simulink model "pfb_fft_d3a"  (R2021a)
settings: Solver=VariableStepAuto  StartTime=0.0  StopTime=100.0  RelTol=1e-3
undefined symbols (not defined in the file): i, pfb_coeff_gen_calc
libraries: xbsIndex_r4 x11529, casper_library_misc x39, casper_library_delays x39, xbsReplacements_r4 x2
(part 40 of 118)

== system pfb_fft_d3a/fft_wideband_real/fft_biplex_real_4x/biplex_core/fft_stage_10/butterfly_direct ==
  a : Inport
  b : Inport  Port=2
  sync_in : Inport  Port=3
  shift : Inport  Port=4
  Concat : xbsIndex_r4/Concat  num_inputs=2  dbl_ovrd=off  block_type=concat
  bus_add : Subsystem  AncestorBlock=casper_library_bus/bus_addsub  mask(bus_addsub){opmode=0, n_bits_a=[18 18], bin_pt_a=17, type_a=1, n_bits_b=[19 19], bin_pt_b=17, type_b=1, cmplx=on, misc=off, async=off, floating_point=off, float_type=single, exp_width=8, frac_width=24, n_bits_out=20, bin_pt_out=17, type_out=1, quantization=0, overflow=0, add_implementation=behavioral HDL, csp_latency=1, pipeline_en=off, pipeline_latency=0}
      mask prompts: opmode "mode (Addition=0, Subtraction=1)"; n_bits_a "a input bit widths"; bin_pt_a "a input binary points"; type_a "a input type (Unsigned=0, Signed=1)"; n_bits_b "b input bit widths"; bin_pt_b "b input binary points"; type_b "b input type (Unsigned=0, Signed=1)"; cmplx "complex"; misc "misc support"; async "asynchronous operation"; floating_point "floating point"; exp_width "exponent width"; frac_width "fraction width"; n_bits_out "output bit widths"; bin_pt_out "output binary points"; type_out "output type (Unsigned=0, Signed=1)"; quantization "quantization strategy (Truncate=0, Round  (unbiased: +/- Inf)=1)"; overflow "overflow strategy (Wrap=0, Saturate=1, Flag as error=2)"; add_implementation "adder implementation"; csp_latency "latency"; pipeline_en "pipeline enable"; pipeline_latency "pipeline latency"
      mask help: Add/subtract components of two busses
      mask init: same as pfb_fft_d3a/fft_wideband_real/fft_direct/butterfly0_0/bus_add
      mask Callback floating_point:
      | onoff = get_param(gcb, 'floating_point');
      | if strcmp(onoff,'on')
      |     enable_fixpt = 'off';
      |     set_param_state(gcb, 'float_type', 'on')
      | 
      |     f_type = get_param(gcb, 'float_type');
      |     if strcmp(f_type,'custom')
      |         set_param_state(gcb, 'exp_width', 'on')
      |         set_param_state(gcb, 'frac_width', 'on')
      |     else
      |         set_param_state(gcb, 'exp_width', 'off')
      |         set_param_state(gcb, 'frac_width', 'off')
      |     end
      | 
      | 
      | else
      |     enable_fixpt = 'on';
      |     set_param_state(gcb, 'float_type', 'off')
      |     set_param_state(gcb, 'exp_width', 'off')
      |     set_param_state(gcb, 'frac_width', 'off')
      | end
      | 
      | set_param_state(gcb, 'n_bits_a', enable_fixpt)
      | set_param_state(gcb, 'bin_pt_a', enable_fixpt)
      | set_param_state(gcb, 'type_a', enable_fixpt)
      | set_param_state(gcb, 'n_bits_b', enable_fixpt)
      | set_param_state(gcb, 'bin_pt_b', enable_fixpt)
      | set_param_state(gcb, 'type_b', enable_fixpt)
      | 
      | set_param_state(gcb, 'n_bits_out', enable_fixpt)
      | set_param_state(gcb, 'bin_pt_out', enable_fixpt)
      | set_param_state(gcb, 'type_out', enable_fixpt)
      | set_param_state(gcb, 'quantization', enable_fixpt)
      | set_param_state(gcb, 'overflow', enable_fixpt)
      mask TypeOptions float_type: single | custom
      mask Callback float_type:
      | f_type = get_param(gcb, 'float_type');
      | if strcmp(f_type,'custom')
      |     set_param_state(gcb, 'exp_width', 'on')
      |     set_param_state(gcb, 'frac_width', 'on')
      | else
      |     set_param_state(gcb, 'exp_width', 'off')
      |     set_param_state(gcb, 'frac_width', 'off')
      | end
      mask TypeOptions add_implementation: behavioral HDL | fabric core | DSP48 core
  bus_convert : Subsystem  AncestorBlock=casper_library_bus/bus_convert  mask(bus_convert){n_bits_in=[21 21 21 21], bin_pt_in=[18 18 18 18], cmplx=on, n_bits_out=18, bin_pt_out=17, quantization=2, overflow=0, csp_latency=conv_latency, of=on, misc=off}
      mask prompts: n_bits_in "input bit widths"; bin_pt_in "input binary points"; cmplx "input complex"; n_bits_out "output bit widths"; bin_pt_out "output binary points"; quantization "quantization strategy (Truncate=0, Round  (unbiased: +/- Inf)=1, Round (unbiased: Even Values)=2)"; overflow "overflow strategy (Wrap=0, Saturate=1, Flag as error=2)"; csp_latency "latency"; of "overflow indication"; misc "misc support"
      mask help: Convert components of busses
      mask init: same as pfb_fft_d3a/fft_wideband_real/fft_direct/butterfly0_0/bus_convert
  bus_expand : Subsystem  AncestorBlock=casper_library_flow_control/bus_expand  mask(bus_expand){mode=divisions of equal size, outputNum=2, outputWidth=[72 72], outputBinaryPt=[0,0], outputArithmeticType=[0,0], show_format=off, outputToWorkspace=off, variablePrefix=out, outputToModelAsWell=on}
      mask prompts: outputNum "Number of outputs:"; outputWidth "Output width:"; outputBinaryPt "Output binary point position:"; outputArithmeticType "Output arithmetic type (ufix=0, fix=1, bool=2):"; show_format "Print format string?"; outputToWorkspace "Output to workspace?"; variablePrefix "Variable name prefix:"; outputToModelAsWell "Output to model as well?"
      mask help:
      | Expands a 'bus' made using a bus_create or Xilinx
      | concat block.
      | The input will be divided into the specified number
      | of outputs with the specified arithmetic types.
      | Divisions are made from most significant bit.
      mask init: same as pfb_fft_d3a/fft_wideband_real/fft_biplex_real_4x/pol0_debus
      settings: AttributesFormatString=2 outputs
      mask TypeOptions mode: divisions of equal size | divisions of arbitrary size
      mask Callback mode: %bus_expand_callback();
      mask Callback outputWidth: %bus_expand_callback();
      mask Callback outputToWorkspace: %bus_expand_callback();
  bus_norm0 : Subsystem  AncestorBlock=casper_library_bus/bus_convert  mask(bus_convert){n_bits_in=[20 20 20 20], bin_pt_in=[17 17 17 17], cmplx=on, n_bits_out=21, bin_pt_out=18, quantization=0, overflow=0, csp_latency=0, of=off, misc=off}
      mask prompts: n_bits_in "input bit widths"; bin_pt_in "input binary points"; cmplx "input complex"; n_bits_out "output bit widths"; bin_pt_out "output binary points"; quantization "quantization strategy (Truncate=0, Round  (unbiased: +/- Inf)=1, Round (unbiased: Even Values)=2)"; overflow "overflow strategy (Wrap=0, Saturate=1, Flag as error=2)"; csp_latency "latency"; of "overflow indication"; misc "misc support"
      mask help: Convert components of busses
      mask init: same as pfb_fft_d3a/fft_wideband_real/fft_direct/butterfly0_0/bus_convert
  bus_norm1 : Subsystem  AncestorBlock=casper_library_bus/bus_convert  mask(bus_convert){n_bits_in=[20 20 20 20], bin_pt_in=[18 18 18 18], cmplx=on, n_bits_out=21, bin_pt_out=18, quantization=0, overflow=0, csp_latency=0, of=off, misc=off}
      mask prompts: n_bits_in "input bit widths"; bin_pt_in "input binary points"; cmplx "input complex"; n_bits_out "output bit widths"; bin_pt_out "output binary points"; quantization "quantization strategy (Truncate=0, Round  (unbiased: +/- Inf)=1, Round (unbiased: Even Values)=2)"; overflow "overflow strategy (Wrap=0, Saturate=1, Flag as error=2)"; csp_latency "latency"; of "overflow indication"; misc "misc support"
      mask help: Convert components of busses
      mask init: same as pfb_fft_d3a/fft_wideband_real/fft_direct/butterfly0_0/bus_convert
  bus_relational : Subsystem  AncestorBlock=casper_library_bus/bus_relational  mask(bus_relational){n_bits_a=4, bin_pt_a=0, type_a=0, n_bits_b=[4 4], bin_pt_b=0, type_b=0, en=off, misc=off, mode=a!=b, csp_latency=1}
      mask prompts: n_bits_a "a input bit widths"; bin_pt_a "a input binary points"; type_a "a input type (Unsigned=0, Signed=1)"; n_bits_b "b input bit widths"; bin_pt_b "b input binary points"; type_b "b input type (Unsigned=0, Signed=1)"; en "en port"; misc "misc support"; mode "comparison:"; csp_latency "latency"
      mask help: Find the relational product of two busses
      mask init: same as pfb_fft_d3a/fft_wideband_real/fft_direct/butterfly0_0/bus_relational
      mask TypeOptions mode: a=b | a!=b | a<b | a>b | a<=b | a>=b
  bus_scale : Subsystem  AncestorBlock=casper_library_bus/bus_scale  mask(bus_scale){n_bits_in=[20 20 20 20], bin_pt_in=17, type_in=1, cmplx=on, scale_factor=-1, misc=off}
      mask prompts: n_bits_in "input bit widths"; bin_pt_in "input binary points"; type_in "input types"; cmplx "input complex"; scale_factor "scale factor (2^?)"; misc "misc support"
      mask help: Convert components of busses
      mask init:
      | bus_scale_init(gcb, ...
      |     'n_bits_in', n_bits_in, ...
      |     'bin_pt_in', bin_pt_in, ...
      |     'type_in', type_in, ...
      |     'cmplx', cmplx, ...
      |     'scale_factor', scale_factor, ...
      |     'misc', misc);
  bus_sub : Subsystem  AncestorBlock=casper_library_bus/bus_addsub  mask(bus_addsub){opmode=1, n_bits_a=[18 18], bin_pt_a=17, type_a=1, n_bits_b=[19 19], bin_pt_b=17, type_b=1, cmplx=on, misc=off, async=off, floating_point=off, float_type=single, exp_width=8, frac_width=24, n_bits_out=20, bin_pt_out=17, type_out=1, quantization=0, overflow=0, add_implementation=behavioral HDL, csp_latency=1, pipeline_en=off, pipeline_latency=0}
      mask prompts: opmode "mode (Addition=0, Subtraction=1)"; n_bits_a "a input bit widths"; bin_pt_a "a input binary points"; type_a "a input type (Unsigned=0, Signed=1)"; n_bits_b "b input bit widths"; bin_pt_b "b input binary points"; type_b "b input type (Unsigned=0, Signed=1)"; cmplx "complex"; misc "misc support"; async "asynchronous operation"; floating_point "floating point"; exp_width "exponent width"; frac_width "fraction width"; n_bits_out "output bit widths"; bin_pt_out "output binary points"; type_out "output type (Unsigned=0, Signed=1)"; quantization "quantization strategy (Truncate=0, Round  (unbiased: +/- Inf)=1)"; overflow "overflow strategy (Wrap=0, Saturate=1, Flag as error=2)"; add_implementation "adder implementation"; csp_latency "latency"; pipeline_en "pipeline enable"; pipeline_latency "pipeline latency"
      mask help: Add/subtract components of two busses
      mask init: same as pfb_fft_d3a/fft_wideband_real/fft_direct/butterfly0_0/bus_add
      mask Callback floating_point:
      | onoff = get_param(gcb, 'floating_point');
      | if strcmp(onoff,'on')
      |     enable_fixpt = 'off';
      |     set_param_state(gcb, 'float_type', 'on')
      | 
      |     f_type = get_param(gcb, 'float_type');
      |     if strcmp(f_type,'custom')
      |         set_param_state(gcb, 'exp_width', 'on')
      |         set_param_state(gcb, 'frac_width', 'on')
      |     else
      |         set_param_state(gcb, 'exp_width', 'off')
      |         set_param_state(gcb, 'frac_width', 'off')
      |     end
      | 
      | 
      | else
      |     enable_fixpt = 'on';
      |     set_param_state(gcb, 'float_type', 'off')
      |     set_param_state(gcb, 'exp_width', 'off')
      |     set_param_state(gcb, 'frac_width', 'off')
      | end
      | 
      | set_param_state(gcb, 'n_bits_a', enable_fixpt)
      | set_param_state(gcb, 'bin_pt_a', enable_fixpt)
      | set_param_state(gcb, 'type_a', enable_fixpt)
      | set_param_state(gcb, 'n_bits_b', enable_fixpt)
      | set_param_state(gcb, 'bin_pt_b', enable_fixpt)
      | set_param_state(gcb, 'type_b', enable_fixpt)
      | 
      | set_param_state(gcb, 'n_bits_out', enable_fixpt)
      | set_param_state(gcb, 'bin_pt_out', enable_fixpt)
      | set_param_state(gcb, 'type_out', enable_fixpt)
      | set_param_state(gcb, 'quantization', enable_fixpt)
      | set_param_state(gcb, 'overflow', enable_fixpt)
      mask TypeOptions float_type: single | custom
      mask Callback float_type:
      | f_type = get_param(gcb, 'float_type');
      | if strcmp(f_type,'custom')
      |     set_param_state(gcb, 'exp_width', 'on')
      |     set_param_state(gcb, 'frac_width', 'on')
      | else
      |     set_param_state(gcb, 'exp_width', 'off')
      |     set_param_state(gcb, 'frac_width', 'off')
      | end
      mask TypeOptions add_implementation: behavioral HDL | fabric core | DSP48 core
  constant : xbsIndex_r4/Constant  const=0  gui_display_data_type=Fixed-point  arith_type=Unsigned  n_bits=4  bin_pt=0  preci_type=Single  exp_width=8  frac_width=24  explicit_period=on  period=1  equ=P=C  opselect=C  inp2=PCIN>>17  opr=+  inp1=P  carry=CIN  dbl_ovrd=off  block_type=constant
  delay0 : xbsIndex_r4/Delay  rst=off  infoeditControl=Selection of Reset will increase slice count due to use of real FFs and instead of SRLs  en=off  latency=add_latency+1+conv_latency  reg_retiming=on  dbl_ovrd=off  block_type=delay
  munge : Subsystem  AncestorBlock=casper_library_flow_control/munge  mask(munge){divisions=4, div_size=[2 2 2 2], order=[0 2 1 3], arith_type_out=Unsigned, bin_pt_out=0}
      mask prompts: divisions "Number of divisions"; div_size "Division size (bits)"; order "Division packing order"; arith_type_out "Output arithmetic type"; bin_pt_out "Output binary point"
      mask help: Splits an input bus into the specified number of divisions and then recombines them in the order specified (most significant division = 0,least = number divisions-1)
      mask init:
      | munge_init(gcb, ...
      |     'divisions', divisions, ...
      |     'div_size', div_size, ...
      |     'order', order, ...
      |     'arith_type_out', arith_type_out, ...
      |     'bin_pt_out', bin_pt_out);
      settings: AttributesFormatString=|
      | split:[2 2 2 2]
      | join:[0 2 1 3]
      | Unsigned [8,0]
      mask TypeOptions arith_type_out: Unsigned | Signed  (2's comp) | Floating-point
  mux : Subsystem  AncestorBlock=casper_library_bus/bus_mux  mask(bus_mux){n_inputs=2, n_bits=[21 21 21 21 21 21 21 21], cmplx=off, misc=off, mux_latency=1}
      mask prompts: n_inputs "number of inputs"; n_bits "input bit widths"; cmplx "complex data"; misc "misc support"; mux_latency "mux latency"
      mask help: Mux components of bus
      mask init:
      | bus_mux_init(gcb, ...
      |     'n_inputs', n_inputs, ...
      |     'n_bits', n_bits, ...
      |     'cmplx', cmplx, ...
      |     'misc', misc, ...
      |     'mux_latency', mux_latency);
  shift_replicate : Subsystem  AncestorBlock=casper_library_bus/bus_replicate  mask(bus_replicate){replication=8, csp_latency=1, misc=off, implementation=core}
      mask prompts: replication "replication factor"; csp_latency "latency"; misc "misc support"; implementation "delay implementation"
      mask help: Output bus formed by replicating input bus a number of times
      mask init:
      | bus_replicate_init(gcb, ...
      |     'replication', replication, ...
      |     'csp_latency', csp_latency, ...
      |     'implementation', implementation, ...
      |     'misc', misc);
      mask TypeOptions implementation: core | behavioral
  twiddle : Subsystem  AncestorBlock=casper_library_ffts_twiddle/twiddle_general  mask(twiddle_general){n_inputs=2, FFTSize=11, Coeffs=[0 1 2 3 4 5 6 7 8 9 10 11 12 13 14 15 16 17 18 19 20 21 22 23 24 25 26 27 28 29 30 31 32 33 34 35 36 37 38 39 40 41 42 43 44 45 46 47 48 49 50 51 52 53 54 55 56 57 58 59 60 61 62 63 64 65 66 67 68 69 70 71 72 73 74 75 76 77 78 79 80 81 82 83 84 85 86 87 88 89 90 91 92 93 94 95 96 97 98 99 100 101 102 103 104 105 106 107 108 109 110 111 112 113 114 115 116 117 118 119 120 121 122 123 124 125 126 127 128 129 130 131 132 133 134 135 136 137 138 139 140 141 142 143 144 145 146 147 148 149 150 151 152 153 154 155 156 157 158 159 160 161 162 163 164 165 166 167 168 169 170 171 172 173 174 175 176 177 178 179 180 181 182 183 184 185 186 187 188 189 190 191 192 193 194 195 196 197 198 199 200 201 202 203 204 205 206 207 208 209 210 211 212 213 214 215 216 217 218 219 220 221 222 223 224 225 226 227 228 229 230 231 232 233 234 235 236 237 238 239 240 241 242 243 244 245 246 247 248 249 250 251 252 253 254 255 256 257 258 259 260 261 262 263 264 265 266 267 268 269 270 271 272 273 274 275 276 277 278 279 280 281 282 283 284 285 286 287 288 289 290 291 292 293 294 295 296 297 298 299 300 301 302 303 304 305 306 307 308 309 310 311 312 313 314 315 316 317 318 319 320 321 322 323 324 325 326 327 328 329 330 331 332 333 334 335 336 337 338 339 340 341 342 343 344 345 346 347 348 349 350 351 352 353 354 355 356 357 358 359 360 361 362 363 364 365 366 367 368 369 370 371 372 373 374 375 376 377 378 379 380 381 382 383 384 385 386 387 388 389 390 391 392 393 394 395 396 397 398 399 400 401 402 403 404 405 406 407 408 409 410 411 412 413 414 415 416 417 418 419 420 421 422 423 424 425 426 427 428 429 430 431 432 433 434 435 436 437 438 439 440 441 442 443 444 445 446 447 448 449 450 451 452 453 454 455 456 457 458 459 460 461 462 463 464 465 466 467 468 469 470 471 472 473 474 475 476 477 478 479 480 481 482 483 484 485 486 487 488 489 490 491 492 493 494 495 496 497 498 499 500 501 502 503 504 505 506 507 508 509 510 511], StepPeriod=1, coeff_bit_width=18, input_bit_width=18, bin_pt_in=17, async=off, floating_point=off, float_type=single, exp_width=8, frac_width=24, add_latency=1, mult_latency=2, bram_latency=2, conv_latency=1, add_pipe_latency=0, mult_pipe_latency=0, coeffs_bit_limit=9, coeff_sharing=on, coeff_decimation=on, coeff_generation=off, cal_bits=1, n_bits_rotation=25, max_fanout=4, use_hdl=on, use_embedded=off, quantization=Round  (unbiased: Even Values), overflow=Wrap}
      mask prompts: n_inputs "Number inputs"; FFTSize "FFT Size (2^?)"; Coeffs "Coefficients:"; StepPeriod "Coefficient Step Period (2^?)"; coeff_bit_width "Coefficient Bit Width"; input_bit_width "Input Bit Width"; bin_pt_in "Input binary point"; async "Asynchronous operation"; floating_point "floating point"; float_type "float type"; exp_width "exponent width"; frac_width "fraction width"; add_latency "Add Latency"; mult_latency "Mult Latency"; bram_latency "BRAM Latency"; conv_latency "Convert Latency"; add_pipe_latency "Add Pipeline Latency"; mult_pipe_latency "CMult Pipeline Latency"; coeffs_bit_limit "Number bits above which to store stage's coefficients in BRAM (2^? bits)"; coeff_sharing "BRAM sharing in coeff storage"; coeff_decimation "Store a fraction of coeff factors where useful"; coeff_generation "Generate coeffs with multipliers where useful"; cal_bits "Number calibration locations when generating coeffs (2^?)"; n_bits_rotation "Feedback rotation vector resolution"; max_fanout "Maximum fanout"; use_hdl "Use behavioural HDL for multipliers"; use_embedded "Use embedded multipliers"; quantization "Quantization Behavior"; overflow "Overflow Behavior"
      mask help: Used in biplex pipelined FFT.
      mask init: same as pfb_fft_d3a/fft_wideband_real/fft_direct/butterfly0_0/twiddle
      settings: AttributesFormatString=|
      | data=(18,17)
      | coeffs=(18,17)
      | (Round  (unbiased: Even Values),Wrap)
      mask Callback floating_point:
      | onoff = get_param(gcb, 'floating_point');
      | if strcmp(onoff,'on')
      |     enable_fixpt = 'off';
      |     set_param_state(gcb, 'float_type', 'on')
      | 
      |     f_type = get_param(gcb, 'float_type');
      |     if strcmp(f_type,'custom')
      |         set_param_state(gcb, 'exp_width', 'on')
      |         set_param_state(gcb, 'frac_width', 'on')
      |     else
      |         set_param_state(gcb, 'exp_width', 'off')
      |         set_param_state(gcb, 'frac_width', 'off')
      |     end
      | 
      | 
      | else
      |     enable_fixpt = 'on';
      |     set_param_state(gcb, 'float_type', 'off')
      |     set_param_state(gcb, 'exp_width', 'off')
      |     set_param_state(gcb, 'frac_width', 'off')
      | end
      | 
      | set_param_state(gcb, 'input_bit_width', enable_fixpt)
      | set_param_state(gcb, 'bin_pt_in', enable_fixpt)
      | set_param_state(gcb, 'coeff_bit_width', enable_fixpt)
      mask TypeOptions float_type: single | custom
      mask Callback float_type:
      | f_type = get_param(gcb, 'float_type');
      | if strcmp(f_type,'custom')
      |     set_param_state(gcb, 'exp_width', 'on')
      |     set_param_state(gcb, 'frac_width', 'on')
      | else
      |     set_param_state(gcb, 'exp_width', 'off')
      |     set_param_state(gcb, 'frac_width', 'off')
      | end
      mask Callback use_hdl: twiddle_general_callback(gcb);
      mask TypeOptions quantization: Truncate | Round  (unbiased: +/- Inf) | Round  (unbiased: Even Values)
      mask TypeOptions overflow: Wrap | Saturate | Error
      mask DialogControl ParameterTabVar0 Prompt: Basic
      mask DialogControl ParameterTabVar01 Prompt: Latency
      mask DialogControl ParameterTabVar012 Prompt: Implementation
  a+bw : Outport
  a-bw : Outport  Port=2
  of : Outport  Port=3
  sync_out : Outport  Port=4
  wires:
  a/1 -> twiddle/1(ai)
  b/1 -> twiddle/2(bi)
  sync_in/1 -> twiddle/3(sync_in)
  twiddle/1(ao) -> bus_add/1(a), bus_sub/1(a)
  twiddle/2(bwo) -> bus_add/2(b), bus_sub/2(b)
  bus_add/1(dout) -> Concat/1
  bus_sub/1(dout) -> Concat/2
  shift/1 -> shift_replicate/1(in)
  Concat/1 -> bus_norm0/1(din), bus_scale/1(din)
  bus_scale/1(dout) -> bus_norm1/1(din)
  shift_replicate/1(out) -> mux/1(sel)
  bus_norm0/1(dout) -> mux/2(d0)
  bus_norm1/1(dout) -> mux/3(d1)
  mux/1(out) -> bus_convert/1(din)
  bus_convert/1(dout) -> bus_expand/1(bus_in)
  bus_expand/1(msb_out2) -> a+bw/1
  bus_expand/2(lsb_out1) -> a-bw/1
  bus_convert/2(overflow) -> munge/1(din)
  constant/1 -> bus_relational/1(a)
  munge/1(dout) -> bus_relational/2(b)
  bus_relational/1(a!=b) -> of/1
  twiddle/3(sync_out) -> delay0/1
  delay0/1 -> sync_out/1

== system pfb_fft_d3a/fft_wideband_real/fft_biplex_real_4x/biplex_core/fft_stage_10/delay0 ==
  din : Inport
  del1 : xbsIndex_r4/Delay  rst=off  infoeditControl=Selection of Reset will increase slice count due to use of real FFs and instead of SRLs  en=off  latency=2  reg_retiming=on  dbl_ovrd=off  block_type=delay
  del2 : xbsIndex_r4/Delay  rst=off  infoeditControl=Selection of Reset will increase slice count due to use of real FFs and instead of SRLs  en=off  latency=2  reg_retiming=on  dbl_ovrd=off  block_type=delay
  din_expand : Subsystem  AncestorBlock=casper_library_flow_control/bus_expand  mask(bus_expand){mode=divisions of arbitrary size, outputNum=2, outputWidth=[36  36], outputBinaryPt=[0  0], outputArithmeticType=[0  0], show_format=on, outputToWorkspace=off, variablePrefix=, outputToModelAsWell=on}
      mask prompts: outputNum "Number of outputs:"; outputWidth "Output width:"; outputBinaryPt "Output binary point position:"; outputArithmeticType "Output arithmetic type (ufix=0, fix=1, bool=2):"; show_format "Print format string?"; outputToWorkspace "Output to workspace?"; variablePrefix "Variable name prefix:"; outputToModelAsWell "Output to model as well?"
      mask help:
      | Expands a 'bus' made using a bus_create or Xilinx
      | concat block.
      | The input will be divided into the specified number
      | of outputs with the specified arithmetic types.
      | Divisions are made from most significant bit.
      mask init: same as pfb_fft_d3a/fft_wideband_real/fft_biplex_real_4x/pol0_debus
      settings: AttributesFormatString=2 outputs: uf36.0,uf36.0,
      mask TypeOptions mode: divisions of equal size | divisions of arbitrary size
      mask Callback mode: %bus_expand_callback();
      mask Callback outputWidth: %bus_expand_callback();
      mask Callback outputToWorkspace: %bus_expand_callback();
  dout_compress : Subsystem  AncestorBlock=casper_library_flow_control/bus_create  mask(bus_create){inputNum=2}
      mask prompts: inputNum "Number of inputs:"
      mask init:
      | bus_create_init(gcb,...
      |     'inputNum', inputNum);
  dout : Outport
  wires:
  din/1 -> din_expand/1(bus_in)
  din_expand/1(msb_out2) -> del1/1
  din_expand/2(lsb_out1) -> del2/1
  del1/1 -> dout_compress/1(in1)
  del2/1 -> dout_compress/2(in2)
  dout_compress/1(bus_out) -> dout/1

== system pfb_fft_d3a/fft_wideband_real/fft_biplex_real_4x/biplex_core/fft_stage_10/delay1 ==
  din : Inport
  del1 : xbsIndex_r4/Delay  rst=off  infoeditControl=Selection of Reset will increase slice count due to use of real FFs and instead of SRLs  en=off  latency=2  reg_retiming=on  dbl_ovrd=off  block_type=delay
  del2 : xbsIndex_r4/Delay  rst=off  infoeditControl=Selection of Reset will increase slice count due to use of real FFs and instead of SRLs  en=off  latency=2  reg_retiming=on  dbl_ovrd=off  block_type=delay
  din_expand : Subsystem  AncestorBlock=casper_library_flow_control/bus_expand  mask(bus_expand){mode=divisions of arbitrary size, outputNum=2, outputWidth=[36  36], outputBinaryPt=[0  0], outputArithmeticType=[0  0], show_format=on, outputToWorkspace=off, variablePrefix=, outputToModelAsWell=on}
      mask prompts: outputNum "Number of outputs:"; outputWidth "Output width:"; outputBinaryPt "Output binary point position:"; outputArithmeticType "Output arithmetic type (ufix=0, fix=1, bool=2):"; show_format "Print format string?"; outputToWorkspace "Output to workspace?"; variablePrefix "Variable name prefix:"; outputToModelAsWell "Output to model as well?"
      mask help:
      | Expands a 'bus' made using a bus_create or Xilinx
      | concat block.
      | The input will be divided into the specified number
      | of outputs with the specified arithmetic types.
      | Divisions are made from most significant bit.
      mask init: same as pfb_fft_d3a/fft_wideband_real/fft_biplex_real_4x/pol0_debus
      settings: AttributesFormatString=2 outputs: uf36.0,uf36.0,
      mask TypeOptions mode: divisions of equal size | divisions of arbitrary size
      mask Callback mode: %bus_expand_callback();
      mask Callback outputWidth: %bus_expand_callback();
      mask Callback outputToWorkspace: %bus_expand_callback();
  dout_compress : Subsystem  AncestorBlock=casper_library_flow_control/bus_create  mask(bus_create){inputNum=2}
      mask prompts: inputNum "Number of inputs:"
      mask init:
      | bus_create_init(gcb,...
      |     'inputNum', inputNum);
  dout : Outport
  wires:
  din/1 -> din_expand/1(bus_in)
  din_expand/1(msb_out2) -> del1/1
  din_expand/2(lsb_out1) -> del2/1
  del1/1 -> dout_compress/1(in1)
  del2/1 -> dout_compress/2(in2)
  dout_compress/1(bus_out) -> dout/1

== system pfb_fft_d3a/fft_wideband_real/fft_biplex_real_4x/biplex_core/fft_stage_11/butterfly_direct ==
  a : Inport
  b : Inport  Port=2
  sync_in : Inport  Port=3
  shift : Inport  Port=4
  Concat : xbsIndex_r4/Concat  num_inputs=2  dbl_ovrd=off  block_type=concat
  bus_add : Subsystem  AncestorBlock=casper_library_bus/bus_addsub  mask(bus_addsub){opmode=0, n_bits_a=[18 18], bin_pt_a=17, type_a=1, n_bits_b=[19 19], bin_pt_b=17, type_b=1, cmplx=on, misc=off, async=off, floating_point=off, float_type=single, exp_width=8, frac_width=24, n_bits_out=20, bin_pt_out=17, type_out=1, quantization=0, overflow=0, add_implementation=behavioral HDL, csp_latency=1, pipeline_en=off, pipeline_latency=0}
      mask prompts: opmode "mode (Addition=0, Subtraction=1)"; n_bits_a "a input bit widths"; bin_pt_a "a input binary points"; type_a "a input type (Unsigned=0, Signed=1)"; n_bits_b "b input bit widths"; bin_pt_b "b input binary points"; type_b "b input type (Unsigned=0, Signed=1)"; cmplx "complex"; misc "misc support"; async "asynchronous operation"; floating_point "floating point"; exp_width "exponent width"; frac_width "fraction width"; n_bits_out "output bit widths"; bin_pt_out "output binary points"; type_out "output type (Unsigned=0, Signed=1)"; quantization "quantization strategy (Truncate=0, Round  (unbiased: +/- Inf)=1)"; overflow "overflow strategy (Wrap=0, Saturate=1, Flag as error=2)"; add_implementation "adder implementation"; csp_latency "latency"; pipeline_en "pipeline enable"; pipeline_latency "pipeline latency"
      mask help: Add/subtract components of two busses
      mask init: same as pfb_fft_d3a/fft_wideband_real/fft_direct/butterfly0_0/bus_add
      mask Callback floating_point:
      | onoff = get_param(gcb, 'floating_point');
      | if strcmp(onoff,'on')
      |     enable_fixpt = 'off';
      |     set_param_state(gcb, 'float_type', 'on')
      | 
      |     f_type = get_param(gcb, 'float_type');
      |     if strcmp(f_type,'custom')
      |         set_param_state(gcb, 'exp_width', 'on')
      |         set_param_state(gcb, 'frac_width', 'on')
      |     else
      |         set_param_state(gcb, 'exp_width', 'off')
      |         set_param_state(gcb, 'frac_width', 'off')
      |     end
      | 
      | 
      | else
      |     enable_fixpt = 'on';
      |     set_param_state(gcb, 'float_type', 'off')
      |     set_param_state(gcb, 'exp_width', 'off')
      |     set_param_state(gcb, 'frac_width', 'off')
      | end
      | 
      | set_param_state(gcb, 'n_bits_a', enable_fixpt)
      | set_param_state(gcb, 'bin_pt_a', enable_fixpt)
      | set_param_state(gcb, 'type_a', enable_fixpt)
      | set_param_state(gcb, 'n_bits_b', enable_fixpt)
      | set_param_state(gcb, 'bin_pt_b', enable_fixpt)
      | set_param_state(gcb, 'type_b', enable_fixpt)
      | 
      | set_param_state(gcb, 'n_bits_out', enable_fixpt)
      | set_param_state(gcb, 'bin_pt_out', enable_fixpt)
      | set_param_state(gcb, 'type_out', enable_fixpt)
      | set_param_state(gcb, 'quantization', enable_fixpt)
      | set_param_state(gcb, 'overflow', enable_fixpt)
      mask TypeOptions float_type: single | custom
      mask Callback float_type:
      | f_type = get_param(gcb, 'float_type');
      | if strcmp(f_type,'custom')
      |     set_param_state(gcb, 'exp_width', 'on')
      |     set_param_state(gcb, 'frac_width', 'on')
      | else
      |     set_param_state(gcb, 'exp_width', 'off')
      |     set_param_state(gcb, 'frac_width', 'off')
      | end
      mask TypeOptions add_implementation: behavioral HDL | fabric core | DSP48 core
  bus_convert : Subsystem  AncestorBlock=casper_library_bus/bus_convert  mask(bus_convert){n_bits_in=[21 21 21 21], bin_pt_in=[18 18 18 18], cmplx=on, n_bits_out=18, bin_pt_out=17, quantization=2, overflow=0, csp_latency=conv_latency, of=on, misc=off}
      mask prompts: n_bits_in "input bit widths"; bin_pt_in "input binary points"; cmplx "input complex"; n_bits_out "output bit widths"; bin_pt_out "output binary points"; quantization "quantization strategy (Truncate=0, Round  (unbiased: +/- Inf)=1, Round (unbiased: Even Values)=2)"; overflow "overflow strategy (Wrap=0, Saturate=1, Flag as error=2)"; csp_latency "latency"; of "overflow indication"; misc "misc support"
      mask help: Convert components of busses
      mask init: same as pfb_fft_d3a/fft_wideband_real/fft_direct/butterfly0_0/bus_convert
  bus_expand : Subsystem  AncestorBlock=casper_library_flow_control/bus_expand  mask(bus_expand){mode=divisions of equal size, outputNum=2, outputWidth=[72 72], outputBinaryPt=[0,0], outputArithmeticType=[0,0], show_format=off, outputToWorkspace=off, variablePrefix=out, outputToModelAsWell=on}
      mask prompts: outputNum "Number of outputs:"; outputWidth "Output width:"; outputBinaryPt "Output binary point position:"; outputArithmeticType "Output arithmetic type (ufix=0, fix=1, bool=2):"; show_format "Print format string?"; outputToWorkspace "Output to workspace?"; variablePrefix "Variable name prefix:"; outputToModelAsWell "Output to model as well?"
      mask help:
      | Expands a 'bus' made using a bus_create or Xilinx
      | concat block.
      | The input will be divided into the specified number
      | of outputs with the specified arithmetic types.
      | Divisions are made from most significant bit.
      mask init: same as pfb_fft_d3a/fft_wideband_real/fft_biplex_real_4x/pol0_debus
      settings: AttributesFormatString=2 outputs
      mask TypeOptions mode: divisions of equal size | divisions of arbitrary size
      mask Callback mode: %bus_expand_callback();
      mask Callback outputWidth: %bus_expand_callback();
      mask Callback outputToWorkspace: %bus_expand_callback();
  bus_norm0 : Subsystem  AncestorBlock=casper_library_bus/bus_convert  mask(bus_convert){n_bits_in=[20 20 20 20], bin_pt_in=[17 17 17 17], cmplx=on, n_bits_out=21, bin_pt_out=18, quantization=0, overflow=0, csp_latency=0, of=off, misc=off}
      mask prompts: n_bits_in "input bit widths"; bin_pt_in "input binary points"; cmplx "input complex"; n_bits_out "output bit widths"; bin_pt_out "output binary points"; quantization "quantization strategy (Truncate=0, Round  (unbiased: +/- Inf)=1, Round (unbiased: Even Values)=2)"; overflow "overflow strategy (Wrap=0, Saturate=1, Flag as error=2)"; csp_latency "latency"; of "overflow indication"; misc "misc support"
      mask help: Convert components of busses
      mask init: same as pfb_fft_d3a/fft_wideband_real/fft_direct/butterfly0_0/bus_convert
  bus_norm1 : Subsystem  AncestorBlock=casper_library_bus/bus_convert  mask(bus_convert){n_bits_in=[20 20 20 20], bin_pt_in=[18 18 18 18], cmplx=on, n_bits_out=21, bin_pt_out=18, quantization=0, overflow=0, csp_latency=0, of=off, misc=off}
      mask prompts: n_bits_in "input bit widths"; bin_pt_in "input binary points"; cmplx "input complex"; n_bits_out "output bit widths"; bin_pt_out "output binary points"; quantization "quantization strategy (Truncate=0, Round  (unbiased: +/- Inf)=1, Round (unbiased: Even Values)=2)"; overflow "overflow strategy (Wrap=0, Saturate=1, Flag as error=2)"; csp_latency "latency"; of "overflow indication"; misc "misc support"
      mask help: Convert components of busses
      mask init: same as pfb_fft_d3a/fft_wideband_real/fft_direct/butterfly0_0/bus_convert
  bus_relational : Subsystem  AncestorBlock=casper_library_bus/bus_relational  mask(bus_relational){n_bits_a=4, bin_pt_a=0, type_a=0, n_bits_b=[4 4], bin_pt_b=0, type_b=0, en=off, misc=off, mode=a!=b, csp_latency=1}
      mask prompts: n_bits_a "a input bit widths"; bin_pt_a "a input binary points"; type_a "a input type (Unsigned=0, Signed=1)"; n_bits_b "b input bit widths"; bin_pt_b "b input binary points"; type_b "b input type (Unsigned=0, Signed=1)"; en "en port"; misc "misc support"; mode "comparison:"; csp_latency "latency"
      mask help: Find the relational product of two busses
      mask init: same as pfb_fft_d3a/fft_wideband_real/fft_direct/butterfly0_0/bus_relational
      mask TypeOptions mode: a=b | a!=b | a<b | a>b | a<=b | a>=b
  bus_scale : Subsystem  AncestorBlock=casper_library_bus/bus_scale  mask(bus_scale){n_bits_in=[20 20 20 20], bin_pt_in=17, type_in=1, cmplx=on, scale_factor=-1, misc=off}
      mask prompts: n_bits_in "input bit widths"; bin_pt_in "input binary points"; type_in "input types"; cmplx "input complex"; scale_factor "scale factor (2^?)"; misc "misc support"
      mask help: Convert components of busses
      mask init:
      | bus_scale_init(gcb, ...
      |     'n_bits_in', n_bits_in, ...
      |     'bin_pt_in', bin_pt_in, ...
      |     'type_in', type_in, ...
      |     'cmplx', cmplx, ...
      |     'scale_factor', scale_factor, ...
      |     'misc', misc);
  bus_sub : Subsystem  AncestorBlock=casper_library_bus/bus_addsub  mask(bus_addsub){opmode=1, n_bits_a=[18 18], bin_pt_a=17, type_a=1, n_bits_b=[19 19], bin_pt_b=17, type_b=1, cmplx=on, misc=off, async=off, floating_point=off, float_type=single, exp_width=8, frac_width=24, n_bits_out=20, bin_pt_out=17, type_out=1, quantization=0, overflow=0, add_implementation=behavioral HDL, csp_latency=1, pipeline_en=off, pipeline_latency=0}
      mask prompts: opmode "mode (Addition=0, Subtraction=1)"; n_bits_a "a input bit widths"; bin_pt_a "a input binary points"; type_a "a input type (Unsigned=0, Signed=1)"; n_bits_b "b input bit widths"; bin_pt_b "b input binary points"; type_b "b input type (Unsigned=0, Signed=1)"; cmplx "complex"; misc "misc support"; async "asynchronous operation"; floating_point "floating point"; exp_width "exponent width"; frac_width "fraction width"; n_bits_out "output bit widths"; bin_pt_out "output binary points"; type_out "output type (Unsigned=0, Signed=1)"; quantization "quantization strategy (Truncate=0, Round  (unbiased: +/- Inf)=1)"; overflow "overflow strategy (Wrap=0, Saturate=1, Flag as error=2)"; add_implementation "adder implementation"; csp_latency "latency"; pipeline_en "pipeline enable"; pipeline_latency "pipeline latency"
      mask help: Add/subtract components of two busses
      mask init: same as pfb_fft_d3a/fft_wideband_real/fft_direct/butterfly0_0/bus_add
      mask Callback floating_point:
      | onoff = get_param(gcb, 'floating_point');
      | if strcmp(onoff,'on')
      |     enable_fixpt = 'off';
      |     set_param_state(gcb, 'float_type', 'on')
      | 
      |     f_type = get_param(gcb, 'float_type');
      |     if strcmp(f_type,'custom')
      |         set_param_state(gcb, 'exp_width', 'on')
      |         set_param_state(gcb, 'frac_width', 'on')
      |     else
      |         set_param_state(gcb, 'exp_width', 'off')
      |         set_param_state(gcb, 'frac_width', 'off')
      |     end
      | 
      | 
      | else
      |     enable_fixpt = 'on';
      |     set_param_state(gcb, 'float_type', 'off')
      |     set_param_state(gcb, 'exp_width', 'off')
      |     set_param_state(gcb, 'frac_width', 'off')
      | end
      | 
      | set_param_state(gcb, 'n_bits_a', enable_fixpt)
      | set_param_state(gcb, 'bin_pt_a', enable_fixpt)
      | set_param_state(gcb, 'type_a', enable_fixpt)
      | set_param_state(gcb, 'n_bits_b', enable_fixpt)
      | set_param_state(gcb, 'bin_pt_b', enable_fixpt)
      | set_param_state(gcb, 'type_b', enable_fixpt)
      | 
      | set_param_state(gcb, 'n_bits_out', enable_fixpt)
      | set_param_state(gcb, 'bin_pt_out', enable_fixpt)
      | set_param_state(gcb, 'type_out', enable_fixpt)
      | set_param_state(gcb, 'quantization', enable_fixpt)
      | set_param_state(gcb, 'overflow', enable_fixpt)
      mask TypeOptions float_type: single | custom
      mask Callback float_type:
      | f_type = get_param(gcb, 'float_type');
      | if strcmp(f_type,'custom')
      |     set_param_state(gcb, 'exp_width', 'on')
      |     set_param_state(gcb, 'frac_width', 'on')
      | else
      |     set_param_state(gcb, 'exp_width', 'off')
      |     set_param_state(gcb, 'frac_width', 'off')
      | end
      mask TypeOptions add_implementation: behavioral HDL | fabric core | DSP48 core
  constant : xbsIndex_r4/Constant  const=0  gui_display_data_type=Fixed-point  arith_type=Unsigned  n_bits=4  bin_pt=0  preci_type=Single  exp_width=8  frac_width=24  explicit_period=on  period=1  equ=P=C  opselect=C  inp2=PCIN>>17  opr=+  inp1=P  carry=CIN  dbl_ovrd=off  block_type=constant
  delay0 : xbsIndex_r4/Delay  rst=off  infoeditControl=Selection of Reset will increase slice count due to use of real FFs and instead of SRLs  en=off  latency=add_latency+1+conv_latency  reg_retiming=on  dbl_ovrd=off  block_type=delay
  munge : Subsystem  AncestorBlock=casper_library_flow_control/munge  mask(munge){divisions=4, div_size=[2 2 2 2], order=[0 2 1 3], arith_type_out=Unsigned, bin_pt_out=0}
      mask prompts: divisions "Number of divisions"; div_size "Division size (bits)"; order "Division packing order"; arith_type_out "Output arithmetic type"; bin_pt_out "Output binary point"
      mask help: Splits an input bus into the specified number of divisions and then recombines them in the order specified (most significant division = 0,least = number divisions-1)
      mask init:
      | munge_init(gcb, ...
      |     'divisions', divisions, ...
      |     'div_size', div_size, ...
      |     'order', order, ...
      |     'arith_type_out', arith_type_out, ...
      |     'bin_pt_out', bin_pt_out);
      settings: AttributesFormatString=|
      | split:[2 2 2 2]
      | join:[0 2 1 3]
      | Unsigned [8,0]
      mask TypeOptions arith_type_out: Unsigned | Signed  (2's comp) | Floating-point
  mux : Subsystem  AncestorBlock=casper_library_bus/bus_mux  mask(bus_mux){n_inputs=2, n_bits=[21 21 21 21 21 21 21 21], cmplx=off, misc=off, mux_latency=1}
      mask prompts: n_inputs "number of inputs"; n_bits "input bit widths"; cmplx "complex data"; misc "misc support"; mux_latency "mux latency"
      mask help: Mux components of bus
      mask init:
      | bus_mux_init(gcb, ...
      |     'n_inputs', n_inputs, ...
      |     'n_bits', n_bits, ...
      |     'cmplx', cmplx, ...
      |     'misc', misc, ...
      |     'mux_latency', mux_latency);
  shift_replicate : Subsystem  AncestorBlock=casper_library_bus/bus_replicate  mask(bus_replicate){replication=8, csp_latency=1, misc=off, implementation=core}
      mask prompts: replication "replication factor"; csp_latency "latency"; misc "misc support"; implementation "delay implementation"
      mask help: Output bus formed by replicating input bus a number of times
      mask init:
      | bus_replicate_init(gcb, ...
      |     'replication', replication, ...
      |     'csp_latency', csp_latency, ...
      |     'implementation', implementation, ...
      |     'misc', misc);
      mask TypeOptions implementation: core | behavioral
  twiddle : Subsystem  AncestorBlock=casper_library_ffts_twiddle/twiddle_general  mask(twiddle_general){n_inputs=2, FFTSize=11, Coeffs=[0 1 2 3 4 5 6 7 8 9 10 11 12 13 14 15 16 17 18 19 20 21 22 23 24 25 26 27 28 29 30 31 32 33 34 35 36 37 38 39 40 41 42 43 44 45 46 47 48 49 50 51 52 53 54 55 56 57 58 59 60 61 62 63 64 65 66 67 68 69 70 71 72 73 74 75 76 77 78 79 80 81 82 83 84 85 86 87 88 89 90 91 92 93 94 95 96 97 98 99 100 101 102 103 104 105 106 107 108 109 110 111 112 113 114 115 116 117 118 119 120 121 122 123 124 125 126 127 128 129 130 131 132 133 134 135 136 137 138 139 140 141 142 143 144 145 146 147 148 149 150 151 152 153 154 155 156 157 158 159 160 161 162 163 164 165 166 167 168 169 170 171 172 173 174 175 176 177 178 179 180 181 182 183 184 185 186 187 188 189 190 191 192 193 194 195 196 197 198 199 200 201 202 203 204 205 206 207 208 209 210 211 212 213 214 215 216 217 218 219 220 221 222 223 224 225 226 227 228 229 230 231 232 233 234 235 236 237 238 239 240 241 242 243 244 245 246 247 248 249 250 251 252 253 254 255 256 257 258 259 260 261 262 263 264 265 266 267 268 269 270 271 272 273 274 275 276 277 278 279 280 281 282 283 284 285 286 287 288 289 290 291 292 293 294 295 296 297 298 299 300 301 302 303 304 305 306 307 308 309 310 311 312 313 314 315 316 317 318 319 320 321 322 323 324 325 326 327 328 329 330 331 332 333 334 335 336 337 338 339 340 341 342 343 344 345 346 347 348 349 350 351 352 353 354 355 356 357 358 359 360 361 362 363 364 365 366 367 368 369 370 371 372 373 374 375 376 377 378 379 380 381 382 383 384 385 386 387 388 389 390 391 392 393 394 395 396 397 398 399 400 401 402 403 404 405 406 407 408 409 410 411 412 413 414 415 416 417 418 419 420 421 422 423 424 425 426 427 428 429 430 431 432 433 434 435 436 437 438 439 440 441 442 443 444 445 446 447 448 449 450 451 452 453 454 455 456 457 458 459 460 461 462 463 464 465 466 467 468 469 470 471 472 473 474 475 476 477 478 479 480 481 482 483 484 485 486 487 488 489 490 491 492 493 494 495 496 497 498 499 500 501 502 503 504 505 506 507 508 509 510 511 512 513 514 515 516 517 518 519 520 521 522 523 524 525 526 527 528 529 530 531 532 533 534 535 536 537 538 539 540 541 542 543 544 545 546 547 548 549 550 551 552 553 554 555 556 557 558 559 560 561 562 563 564 565 566 567 568 569 570 571 572 573 574 575 576 577 578 579 580 581 582 583 584 585 586 587 588 589 590 591 592 593 594 595 596 597 598 599 600 601 602 603 604 605 606 607 608 609 610 611 612 613 614 615 616 617 618 619 620 621 622 623 624 625 626 627 628 629 630 631 632 633 634 635 636 637 638 639 640 641 642 643 644 645 646 647 648 649 650 651 652 653 654 655 656 657 658 659 660 661 662 663 664 665 666 667 668 669 670 671 672 673 674 675 676 677 678 679 680 681 682 683 684 685 686 687 688 689 690 691 692 693 694 695 696 697 698 699 700 701 702 703 704 705 706 707 708 709 710 711 712 713 714 715 716 717 718 719 720 721 722 723 724 725 726 727 728 729 730 731 732 733 734 735 736 737 738 739 740 741 742 743 744 745 746 747 748 749 750 751 752 753 754 755 756 757 758 759 760 761 762 763 764 765 766 767 768 769 770 771 772 773 774 775 776 777 778 779 780 781 782 783 784 785 786 787 788 789 790 791 792 793 794 795 796 797 798 799 800 801 802 803 804 805 806 807 808 809 810 811 812 813 814 815 816 817 818 819 820 821 822 823 824 825 826 827 828 829 830 831 832 833 834 835 836 837 838 839 840 841 842 843 844 845 846 847 848 849 850 851 852 853 854 855 856 857 858 859 860 861 862 863 864 865 866 867 868 869 870 871 872 873 874 875 876 877 878 879 880 881 882 883 884 885 886 887 888 889 890 891 892 893 894 895 896 897 898 899 900 901 902 903 904 905 906 907 908 909 910 911 912 913 914 915 916 917 918 919 920 921 922 923 924 925 926 927 928 929 930 931 932 933 934 935 936 937 938 939 940 941 942 943 944 945 946 947 948 949 950 951 952 953 954 955 956 957 958 959 960 961 962 963 964 965 966 967 968 969 970 971 972 973 974 975 976 977 978 979 980 981 982 983 984 985 986 987 988 989 990 991 992 993 994 995 996 997 998 999 1000 1001 1002 1003 1004 1005 1006 1007 1008 1009 1010 1011 1012 1013 1014 1015 1016 1017 1018 1019 1020 1021 1022 1023], StepPeriod=0, coeff_bit_width=18, input_bit_width=18, bin_pt_in=17, async=off, floating_point=off, float_type=single, exp_width=8, frac_width=24, add_latency=1, mult_latency=2, bram_latency=2, conv_latency=1, add_pipe_latency=0, mult_pipe_latency=0, coeffs_bit_limit=9, coeff_sharing=on, coeff_decimation=on, coeff_generation=off, cal_bits=1, n_bits_rotation=25, max_fanout=4, use_hdl=on, use_embedded=off, quantization=Round  (unbiased: Even Values), overflow=Wrap}
      mask prompts: n_inputs "Number inputs"; FFTSize "FFT Size (2^?)"; Coeffs "Coefficients:"; StepPeriod "Coefficient Step Period (2^?)"; coeff_bit_width "Coefficient Bit Width"; input_bit_width "Input Bit Width"; bin_pt_in "Input binary point"; async "Asynchronous operation"; floating_point "floating point"; float_type "float type"; exp_width "exponent width"; frac_width "fraction width"; add_latency "Add Latency"; mult_latency "Mult Latency"; bram_latency "BRAM Latency"; conv_latency "Convert Latency"; add_pipe_latency "Add Pipeline Latency"; mult_pipe_latency "CMult Pipeline Latency"; coeffs_bit_limit "Number bits above which to store stage's coefficients in BRAM (2^? bits)"; coeff_sharing "BRAM sharing in coeff storage"; coeff_decimation "Store a fraction of coeff factors where useful"; coeff_generation "Generate coeffs with multipliers where useful"; cal_bits "Number calibration locations when generating coeffs (2^?)"; n_bits_rotation "Feedback rotation vector resolution"; max_fanout "Maximum fanout"; use_hdl "Use behavioural HDL for multipliers"; use_embedded "Use embedded multipliers"; quantization "Quantization Behavior"; overflow "Overflow Behavior"
      mask help: Used in biplex pipelined FFT.
      mask init: same as pfb_fft_d3a/fft_wideband_real/fft_direct/butterfly0_0/twiddle
      settings: AttributesFormatString=|
      | data=(18,17)
      | coeffs=(18,17)
      | (Round  (unbiased: Even Values),Wrap)
      mask Callback floating_point:
      | onoff = get_param(gcb, 'floating_point');
      | if strcmp(onoff,'on')
      |     enable_fixpt = 'off';
      |     set_param_state(gcb, 'float_type', 'on')
      | 
      |     f_type = get_param(gcb, 'float_type');
      |     if strcmp(f_type,'custom')
      |         set_param_state(gcb, 'exp_width', 'on')
      |         set_param_state(gcb, 'frac_width', 'on')
      |     else
      |         set_param_state(gcb, 'exp_width', 'off')
      |         set_param_state(gcb, 'frac_width', 'off')
      |     end
      | 
      | 
      | else
      |     enable_fixpt = 'on';
      |     set_param_state(gcb, 'float_type', 'off')
      |     set_param_state(gcb, 'exp_width', 'off')
      |     set_param_state(gcb, 'frac_width', 'off')
      | end
      | 
      | set_param_state(gcb, 'input_bit_width', enable_fixpt)
      | set_param_state(gcb, 'bin_pt_in', enable_fixpt)
      | set_param_state(gcb, 'coeff_bit_width', enable_fixpt)
      mask TypeOptions float_type: single | custom
      mask Callback float_type:
      | f_type = get_param(gcb, 'float_type');
      | if strcmp(f_type,'custom')
      |     set_param_state(gcb, 'exp_width', 'on')
      |     set_param_state(gcb, 'frac_width', 'on')
      | else
      |     set_param_state(gcb, 'exp_width', 'off')
      |     set_param_state(gcb, 'frac_width', 'off')
      | end
      mask Callback use_hdl: twiddle_general_callback(gcb);
      mask TypeOptions quantization: Truncate | Round  (unbiased: +/- Inf) | Round  (unbiased: Even Values)
      mask TypeOptions overflow: Wrap | Saturate | Error
      mask DialogControl ParameterTabVar0 Prompt: Basic
      mask DialogControl ParameterTabVar01 Prompt: Latency
      mask DialogControl ParameterTabVar012 Prompt: Implementation
  a+bw : Outport
  a-bw : Outport  Port=2
  of : Outport  Port=3
  sync_out : Outport  Port=4
  wires:
  a/1 -> twiddle/1(ai)
  b/1 -> twiddle/2(bi)
  sync_in/1 -> twiddle/3(sync_in)
  twiddle/1(ao) -> bus_add/1(a), bus_sub/1(a)
  twiddle/2(bwo) -> bus_add/2(b), bus_sub/2(b)
  bus_add/1(dout) -> Concat/1
  bus_sub/1(dout) -> Concat/2
  shift/1 -> shift_replicate/1(in)
  Concat/1 -> bus_norm0/1(din), bus_scale/1(din)
  bus_scale/1(dout) -> bus_norm1/1(din)
  shift_replicate/1(out) -> mux/1(sel)
  bus_norm0/1(dout) -> mux/2(d0)
  bus_norm1/1(dout) -> mux/3(d1)
  mux/1(out) -> bus_convert/1(din)
  bus_convert/1(dout) -> bus_expand/1(bus_in)
  bus_expand/1(msb_out2) -> a+bw/1
  bus_expand/2(lsb_out1) -> a-bw/1
  bus_convert/2(overflow) -> munge/1(din)
  constant/1 -> bus_relational/1(a)
  munge/1(dout) -> bus_relational/2(b)
  bus_relational/1(a!=b) -> of/1
  twiddle/3(sync_out) -> delay0/1
  delay0/1 -> sync_out/1
